simulink library "gridnode"  (R2025b)
settings: Solver=VariableStepAuto  StartTime=0.0  StopTime=10.0  RelTol=1e-3
settings Model: Creator=jjha  LastModifiedBy=jjha

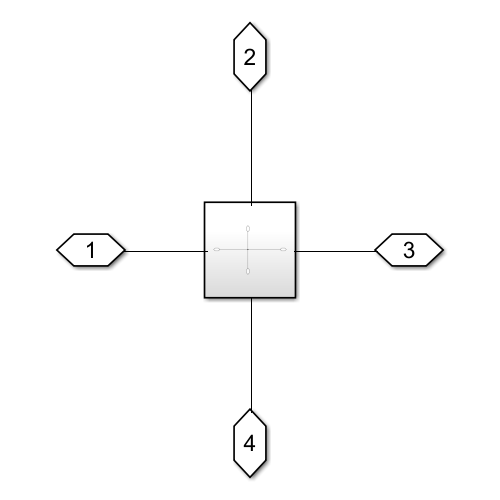
[thumbnail: Simulink's stored preview of the top-level diagram]
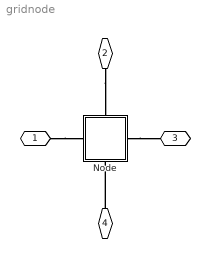
== system gridnode ==
  Node : Subsystem
      settings: PortSchema="{\"entries\":[{\"content\":{\"sides\":[{\"content\":{\"connectorIds\":[\"LConn1\"]},\"type\":\"ConnectorPlacement.EquallySpacedRectSide\",\"uuid\":\"ea590e09-5d16-49b2-923f-8461aff6ddfe\"},{\"content\":{\"connectorIds\":[\"RConn1\"],\"side\":\"RIGHT\"},\"type\":\"ConnectorPlacement.EquallySpacedRectSide\",\"uuid\":\"a78871b9-45b2-474e-98e4-a986e9414988\"},{\"content\":{\"connectorIds\":[\"LConn2\"],\"side\":\"TOP\"},\"type\":\"ConnectorPlacement.EquallySpacedRectSide\",\"uuid\":\"9d9268e9-b8dc-43c2-a54e-8a790b0e4fd5\"},{\"content\":{\"connectorIds\":[\"RConn2\"],\"side\":\"BOTTOM\"},\"type\":\"ConnectorPlacement.EquallySpacedRectSide\",\"uuid\":\"2e3983c1-208b-474c-9b64-be0bde301adf\"}]},\"type\":\"ConnectorPlacement.EquallySpacedConnector\",\"uuid\":\"fda160ea-3140-4f7a-b3cb-ce9d21df8ebe\"}],\"packageUris\":[\"http://schema.mathworks.com/mf0/Connector/R2020b\"],\"version\":\"1.0\"}"
  "   " : PMIOPort  Side=Left
  " " : PMIOPort  Port=2  Side=Left
  "  " : PMIOPort  Port=3  Side=Right
  "    " : PMIOPort  Port=4  Side=Right
  connections:
  "   "/RConn1 -- Node/LConn1
  " "/RConn1 -- Node/LConn2
  Node/RConn1 -- "  "/RConn1
  "    "/RConn1 -- Node/RConn2

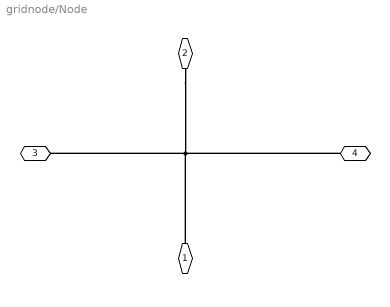
== system gridnode/Node ==
  "   " : PMIOPort  Side=Left
  " " : PMIOPort  Port=2  Side=Left
  "  " : PMIOPort  Port=3  Side=Right
  "    " : PMIOPort  Port=4  Side=Right
  connections:
  "   "/RConn1 -- "    "/RConn1 -- " "/RConn1 -- "  "/RConn1
